simulink model "main_simulation_MM"  (R2025b)
settings: Solver=VariableStepAuto  StartTime=0.0  StopTime=inf  FixedStep=0.001  RelTol=1e-3  EnableMultiTasking=on
values from neighbouring files (symbols this model uses):
  m = 'main_simulation_MM'    [patanahikyahaiyeh.m]    (also in patanahikyahaiyeh2.m)
  s = get_param(ln,'SrcPortHandle')    [patanahikyahaiyeh2.m]
undefined symbols (not defined in the file or in its folder): X, Y, Z
libraries: sm_lib x115, nesl_utility x18, quarc_library x1
(part 3 of 3)

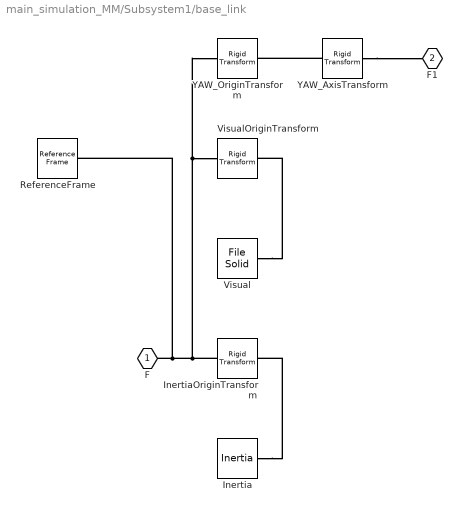
== system main_simulation_MM/Subsystem1/base_link ==
  Inertia : sm_lib/Body Elements/Inertia  InertiaType=Custom  Mass=3.89847036294307  MassUnits=kg  CenterOfMass=[0, 0, 0]  CenterOfMassUnits=m  MomentsOfInertia=[0.0259717926187233, 0.0237418182185852, 0.048730018421969]  MomentsOfInertiaUnits=kg*m^2  ProductsOfInertia=[6.90408382921997e-11, -9.203274302752861e-08, 7.41706820354147e-07]  ProductsOfInertiaUnits=kg*m^2  GraphicType=None  MarkerShape=Inertia  MarkerSize=20  GraphicVisPropType=SimpleVisualProperties  GraphicDiffuseColor=[0.5 0.5 0.5]  GraphicOpacity=1  GraphicSpecularColor=[0.5 0.5 0.5 1.0]  GraphicAmbientColor=[0.15 0.15 0.15 1.0]  GraphicEmissiveColor=[0.0 0.0 0.0 1.0]  GraphicShininess=75
  InertiaOriginTransform : sm_lib/Frames and Transforms/Rigid Transform  RotationMethod=RotationSequence  FollAlignAxisA=+X  BaseAlignAxisA=+Y  FollAlignAxisB=+Y  BaseAlignAxisB=+Z  RotationStandardAxis=+Z  RotationAngle=0  RotationAngleUnits=deg  RotationArbitraryAxis=[0 0 1]  RotationSequenceAxes=BaseAxes  RotationSequence=XYZ  RotationSequenceAngles=[0, 0, 0]  RotationSequenceAnglesUnits=rad  RotationMatrix=[1 0 0;0 1 0;0 0 1]  Quaternion=[1 0 0 0]  TranslationMethod=Cartesian  TranslationCartesianOffset=[0.000529200576288575, -2.23307396420992e-06, 0.0267852902177001]  TranslationCartesianOffsetUnits=m  TranslationStandardAxis=+Z  TranslationStandardOffset=0  TranslationStandardOffsetUnits=m  TranslationROffset=0  TranslationROffsetUnits=m  TranslationThetaOffset=0  TranslationThetaOffsetUnits=deg  TranslationZOffset=0  TranslationZOffsetUnits=m
  ReferenceFrame : sm_lib/Frames and Transforms/Reference Frame
  Visual : sm_lib/Body Elements/File Solid  ExtGeomFileName=E:\Projects\Controller Mobile Manipulator\src\qarm\meshes\base_link.STL  UnitType=Custom  ExtGeomFileUnits=m  StepReaderType=HEX  ExportConvexHullGeometry=off  InertiaType=Custom  BasedOnType=DensityFromFile  Density=1000  DensityUnits=kg/m^3  Mass=0  MassUnits=kg  CenterOfMass=[0, 0, 0]  CenterOfMassUnits=m  MomentsOfInertia=[0, 0, 0]  MomentsOfInertiaUnits=kg*m^2  ProductsOfInertia=[0, 0, 0]  ProductsOfInertiaUnits=kg*m^2  GraphicType=FromGeometry  MarkerShape=Sphere  MarkerSize=10  GraphicVisPropType=SimpleVisualProperties  GraphicDiffuseColor=[0.752941176470588, 0.752941176470588, 0.752941176470588]  GraphicOpacity=1  GraphicSpecularColor=[0.5 0.5 0.5 1.0]  GraphicAmbientColor=[0.15 0.15 0.15 1.0]  GraphicEmissiveColor=[0.0 0.0 0.0 1.0]  GraphicShininess=75  DoExposeReferenceFrame=on  SerializedFrames=<Frames/>
  VisualOriginTransform : sm_lib/Frames and Transforms/Rigid Transform  RotationMethod=RotationSequence  FollAlignAxisA=+X  BaseAlignAxisA=+Y  FollAlignAxisB=+Y  BaseAlignAxisB=+Z  RotationStandardAxis=+Z  RotationAngle=0  RotationAngleUnits=deg  RotationArbitraryAxis=[0 0 1]  RotationSequenceAxes=BaseAxes  RotationSequence=XYZ  RotationSequenceAngles=[0, 0, 0]  RotationSequenceAnglesUnits=rad  RotationMatrix=[1 0 0;0 1 0;0 0 1]  Quaternion=[1 0 0 0]  TranslationMethod=Cartesian  TranslationCartesianOffset=[0, 0, 0]  TranslationCartesianOffsetUnits=m  TranslationStandardAxis=+Z  TranslationStandardOffset=0  TranslationStandardOffsetUnits=m  TranslationROffset=0  TranslationROffsetUnits=m  TranslationThetaOffset=0  TranslationThetaOffsetUnits=deg  TranslationZOffset=0  TranslationZOffsetUnits=m
  YAW_AxisTransform : sm_lib/Frames and Transforms/Rigid Transform  RotationMethod=ArbitraryAxis  FollAlignAxisA=+X  BaseAlignAxisA=+Y  FollAlignAxisB=+Y  BaseAlignAxisB=+Z  RotationStandardAxis=+Z  RotationAngle=0  RotationAngleUnits=rad  RotationArbitraryAxis=[1, 0, 0]  RotationSequenceAxes=FollowerAxes  RotationSequence=XYX  RotationSequenceAngles=[0 0 0]  RotationSequenceAnglesUnits=deg  RotationMatrix=[1 0 0;0 1 0;0 0 1]  Quaternion=[1 0 0 0]  TranslationMethod=Cartesian  TranslationCartesianOffset=[0, 0, 0]  TranslationCartesianOffsetUnits=m  TranslationStandardAxis=+Z  TranslationStandardOffset=0  TranslationStandardOffsetUnits=m  TranslationROffset=0  TranslationROffsetUnits=m  TranslationThetaOffset=0  TranslationThetaOffsetUnits=deg  TranslationZOffset=0  TranslationZOffsetUnits=m
  YAW_OriginTransform : sm_lib/Frames and Transforms/Rigid Transform  RotationMethod=RotationSequence  FollAlignAxisA=+X  BaseAlignAxisA=+Y  FollAlignAxisB=+Y  BaseAlignAxisB=+Z  RotationStandardAxis=+Z  RotationAngle=0  RotationAngleUnits=deg  RotationArbitraryAxis=[0 0 1]  RotationSequenceAxes=BaseAxes  RotationSequence=XYZ  RotationSequenceAngles=[0, 0, 0]  RotationSequenceAnglesUnits=rad  RotationMatrix=[1 0 0;0 1 0;0 0 1]  Quaternion=[1 0 0 0]  TranslationMethod=Cartesian  TranslationCartesianOffset=[0, 0, 0]  TranslationCartesianOffsetUnits=m  TranslationStandardAxis=+Z  TranslationStandardOffset=0  TranslationStandardOffsetUnits=m  TranslationROffset=0  TranslationROffsetUnits=m  TranslationThetaOffset=0  TranslationThetaOffsetUnits=deg  TranslationZOffset=0  TranslationZOffsetUnits=m
  F : PMIOPort  Side=Left
  F1 : PMIOPort  Port=2  Side=Right
  connections:
  Inertia/RConn1 -- InertiaOriginTransform/RConn1
  ReferenceFrame/RConn1 -- InertiaOriginTransform/LConn1 -- VisualOriginTransform/LConn1 -- YAW_OriginTransform/LConn1 -- F/RConn1
  Visual/RConn1 -- VisualOriginTransform/RConn1
  YAW_AxisTransform/RConn1 -- F1/RConn1
  YAW_AxisTransform/LConn1 -- YAW_OriginTransform/RConn1

== matlab function main_simulation_MM/Desired Path ==
  data: y output
function y = coordinates()
a = 1.0;                      % half-width of the loop (m)
N = 500;                      % number of waypoints
t = linspace(0, 2*pi, N)';
d = 1 + sin(t).^2;

x  = a*cos(t)./d;
yy = a*sin(t).*cos(t)./d;

% Analytic tangent of the path, used for the heading
dx = -a*sin(t).*(3 - sin(t).^2)./d.^2;
dy =  a*(cos(2*t).*d - 2*sin(t).^2.*cos(t).^2)./d.^2;

% Heading (rad), unwrapped so it never jumps by 2*pi
psi = unwrap(atan2(dy, dx));

y = [x, yy, psi];             % [x y yaw], N-by-3 (yaw drives the planar joint's Rz)
end

== stateflow chart main_simulation_MM/Chart ==
  state PickObject
    entry:
    phase = 0;
    tEnter = tClk;
    during:
    [left_w, right_w, x, y, z, isDone] = MissionPlanner(coordinates_base, tClk, phase, tEnter);
    [qarm_mode, arm_pos, arm_pwm] = controlQArmMode(uint8(0), target_pickup_pos, zero_voltages);
  state Trace
    entry:
    phase = 1;
    tEnter = tClk;
    during:
    [left_w, right_w, x, y, z, isDone] = MissionPlanner(coordinates_base, tClk, phase, tEnter);
    [qarm_mode, arm_pos, arm_pwm] = controlQArmMode(uint8(1), tuck_pos, zero_voltages);
  state DropObject
    entry:
    phase = 2;
    tEnter = tClk;
    count = count + 1;
    during:
    [left_w, right_w, x, y, z, isDone] = MissionPlanner(coordinates_base, tClk, phase, tEnter);
    [qarm_mode, arm_pos, arm_pwm] = controlQArmMode(uint8(2), target_drop_pos, zero_voltages);
  (default) -> PickObject : {count = 0; isDone = 0;}
  Trace -> PickObject [order 1] : [count == lap && (tClk - tEnter >= drop_timeout)]
  PickObject -> Trace : [tClk - tEnter >= 3.0 || arm_attached_sensor == 1]
  DropObject -> Trace : [count < lap && (tClk - tEnter >= drop_timeout)]
  Trace -> DropObject [order 2] : [isDone == 1]
  data: path_points function_input; time function_input; phase function_input; tEnter function_input; left_w function_output; right_w function_output; x function_output; y function_output; z function_output; isDone function_output; qarm_mode function_output; arm_pos function_output; task_phase function_input; target_pos function_input; arm_pwm function_output; override_voltages function_input; tClk input; ChartMode local Enum: ChartModeType; lap input; count local; coordinates_base input; arm_attached_sensor input; drop_timeout input; target_drop_pos input; target_pickup_pos input; tuck_pos input; zero_voltages input; x output; y output; z output; tEnter local; phase local; isDone local; left_w output; right_w output; arm_pos output; arm_pwm output; qarm_mode output
  function [left_w, right_w, x, y, z, isDone] = MissionPlanner(path_points, time, phase, tEnter):
    | function [left_w, right_w, x, y, z, isDone] = MissionPlanner(path_points, time, phase, tEnter)
    |     % left_w / right_w = [dirn, speed] (dirn = +1 forward, -1 reverse)
    |     
    |     b = 0.235;    % wheel track width (m)
    |     v_ref = 0.2;  % forward speed (m/s)
    |     
    |     % Initialize outputs
    |     left_w  = [0, 0];
    |     right_w = [0, 0];
    |     x = path_points(1, 1);
    |     y = path_points(1, 2);
    |     z = path_points(1, 3);
    |     isDone = 0;   % 0 = tracking, 1 = completed lap
    |     
    |     if phase ~= 1
    |         return; % Settle: hold still
    |     end
    |     
    |     tp = max(time - tEnter, 0);
    |     N = size(path_points, 1);
    |     seg = path_points(2:end,:) - path_points(1:end-1,:);
    |     len = sqrt(sum(seg.^2, 2));
    |     cum = [0; cumsum(len)];
    |     
    |     % Target distance traveled along the path
    |     d_target = v_ref * tp; 
    |     
    |     % k = sum(cum <= d_target);
    |     k = 1;
    |     while (k < N-1) && (cum(k+1) <= d_target)
    |         k = k + 1;
    |     end
    |     % Check if the end of the path has been reached
    |     if k > N-2
    |         x = path_points(end, 1);
    |         y = path_points(end, 2);
    |         z = path_points(end, 3);
    |         isDone = 1; % Signal Stateflow that the lap is fully complete!
    |         return; 
    |     end
    |     
    |     % Compute current tracking position (x, y, z) using interpolation
    |     d_rem = d_target - cum(k);   % Distance traveled inside the current segment
    |     ratio = d_rem / len(k);
    |     
    |     x = path_points(k, 1) + ratio * seg(k, 1);
    |     y = path_points(k, 2) + ratio * seg(k, 2);
    |     z = path_points(k, 3) + ratio * seg(k, 3);
    |     
    |     % Calculate wheel velocities
    |     h1 = atan2(seg(k,2), seg(k,1));
    |     h2 = atan2(seg(k+1,2), seg(k+1,1));
    |     dh = atan2(sin(h2-h1), cos(h2-h1));
    |     
    |     omega = dh / (len(k) / v_ref);
    |     
    |     vL = v_ref - omega*b/2;
    |     vR = v_ref + omega*b/2;
    |     
    |     left_w = [2*(vL >= 0) - 1, abs(vL/0.05)];
    |     right_w = [2*(vR >= 0) - 1, abs(vR/0.05)];
    | end
  function [qarm_mode, arm_pos, arm_pwm] = controlQArmMode(task_phase, target_pos, override_voltages):
    | function [qarm_mode, arm_pos, arm_pwm] = controlQArmMode(task_phase, target_pos, override_voltages)
    |     % task_phase: 0 = Pick, 1 = Trace, 2 = Drop
    |     
    |     qarm_mode = uint8(1); 
    |     arm_pwm = zeros(4,1);
    |     
    |     % Hardcoded smooth initial states to prevent t=0 crash
    |     persistent current_arm_state;
    |     if isempty(current_arm_state)
    |         current_arm_state = [0.0; 0.26; -0.52; 0.0]; % Matches tuck_pos initial state
    |     end
    |     
    |     % Enforce correct 4x1 dimensions
    |     target_cmd = target_pos(:);
    |     
    |     % Rate limiter filter: Limit joint movement per time step
    |     % Prevents changes faster than ~1.5 rad/sec
    |     max_step = 1.5 * 0.01; % (Speed limit * fixed time step)
    |     for i = 1:4
    |         error_val = target_cmd(i) - current_arm_state(i);
    |         if abs(error_val) > max_step
    |             current_arm_state(i) = current_arm_state(i) + sign(error_val) * max_step;
    |         else
    |             current_arm_state(i) = target_cmd(i);
    |         end
    |     end
    |     
    |     arm_pos = current_arm_state;
    | end
